simulink model "Frequency_modulation"  (R2025a)
settings: Solver=VariableStepAuto  StartTime=0.0  StopTime=10.0  RelTol=1e-3
libraries: dspfdesign x1, dspsrcs4 x1
settings Model: Creator=Aman  LastModifiedBy=Aman

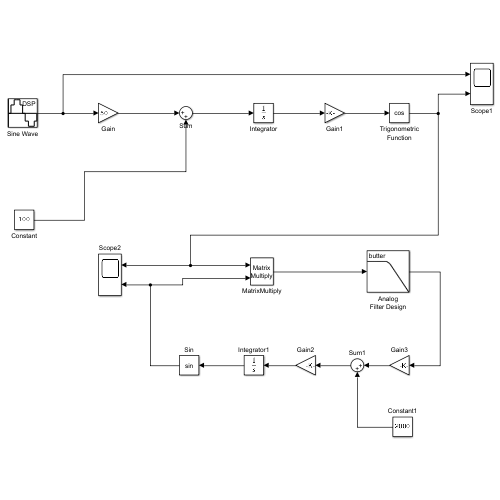
[thumbnail: Simulink's stored preview of the top-level diagram]
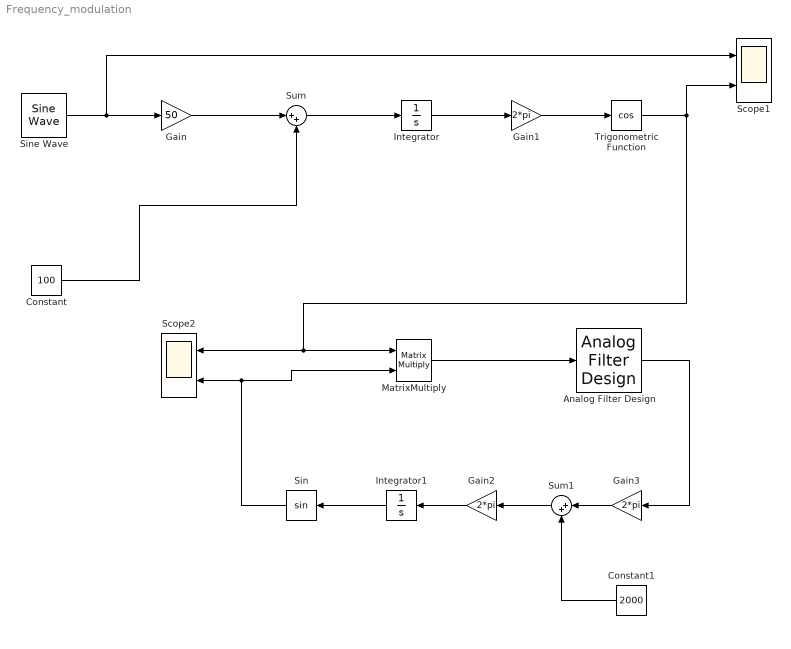
== system Frequency_modulation ==
  Analog Filter Design : dspfdesign/Analog Filter Design  method=Butterworth  filttype=Lowpass  N=5  Wlo=2*pi*10  Whi=80  Rp=2  Rs=40
  Constant : Constant  Value=100
  Constant1 : Constant  Value=2000
  Gain : Gain  Gain=50
  Gain1 : Gain  Gain=2*pi
  Gain2 : Gain  Gain=2*pi
  Gain3 : Gain  Gain=2*pi
  Integrator : Integrator
  Integrator1 : Integrator
  MatrixMultiply : Product  Multiplication=Matrix(*)
  Scope1 : Scope  NumInputPorts=2
      settings: ActiveDisplayYMinimum=-1.25  ActiveDisplayYMaximum=1.25
  Scope2 : Scope  NumInputPorts=2
      settings: ActiveDisplayYMinimum=-1.2499993723920089  ActiveDisplayYMaximum=1.2499999302657787
  Sin : Trigonometry
  Sine Wave : dspsrcs4/Sine Wave  Amplitude=1  Frequency=10  Phase=0  SampleMode=Discrete  OutComplex=Real  CompMethod=Trigonometric fcn  TableSize=Speed  SampleTime=1/1000  SamplesPerFrame=1  ResetState=Restart at time zero  OutputFrames=off  dataType=double  wordLen=16  udDataType=sfix(16)  fracBitsMode=Best precision  numFracBits=15  OutDataTypeStr=double  LastOutDataTypeStr=double
  Sum : Sum  Inputs=|++
  Sum1 : Sum  Inputs=|++
  Trigonometric Function : Trigonometry  Operator=cos
  wires:
  Sine Wave/1 -> Scope1/1, Gain/1
  Gain/1 -> Sum/1
  Sum/1 -> Integrator/1
  Integrator/1 -> Gain1/1
  Gain1/1 -> Trigonometric Function/1
  Constant/1 -> Sum/2
  MatrixMultiply/1 -> Analog Filter Design/1
  Trigonometric Function/1 -> Scope2/1, MatrixMultiply/1, Scope1/2
  Analog Filter Design/1 -> Gain3/1
  Gain3/1 -> Sum1/1
  Sum1/1 -> Gain2/1
  Gain2/1 -> Integrator1/1
  Integrator1/1 -> Sin/1
  Sin/1 -> MatrixMultiply/2, Scope2/2
  Constant1/1 -> Sum1/2
